simulink model "BrakeController_MBD"  (R2021b)
settings: Solver=FixedStepAuto  StartTime=0.0  StopTime=10.0  FixedStep=Ts  RelTol=1e-3
model workspace (MAT data in the model file):
  BrakePressure_Max = Simulink.Parameter
  BrakePressure_Max.Value = 100
  BrakePressure_Max.DataType = 'auto'
  BrakePressure_Max.Complexity = 'real'
  BrakePressure_Max.Dimensions = [1 1]
  Ts = Simulink.Parameter
  Ts.Value = 0.01
  Ts.DataType = 'auto'
  Ts.Complexity = 'real'
  Ts.Dimensions = [1 1]
  k = Simulink.Parameter
  k.Value = 2
  k.DataType = 'auto'
  k.Complexity = 'real'
  k.Dimensions = [1 1]
undefined symbols (not defined in the file): BrakeRequest, VehicleSpeed
settings Model: Creator=QNH2KOR  LastModifiedBy=QNH2KOR

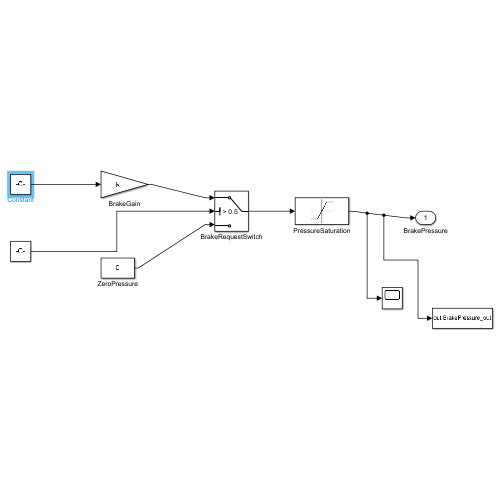
[thumbnail: Simulink's stored preview of the top-level diagram]
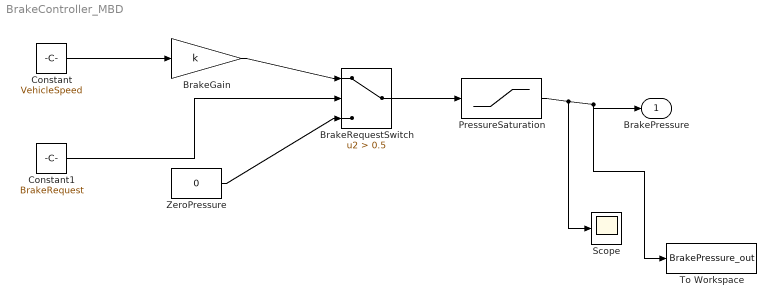
== system BrakeController_MBD ==
  BrakeGain : Gain  Gain=k
  BrakeRequestSwitch : Switch  Criteria=u2 > Threshold  Threshold=0.5
  Constant : Constant  Value=VehicleSpeed
  Constant1 : Constant  Value=BrakeRequest
  PressureSaturation : Saturate  UpperLimit=BrakePressure_Max  LowerLimit=0
  Scope : Scope
  To Workspace : ToWorkspace  VariableName=BrakePressure_out  SaveFormat=Timeseries  SampleTime=-1
  ZeroPressure : Constant  Value=0
  BrakePressure : Outport
  wires:
  Constant/1 -> BrakeGain/1
  BrakeGain/1 -> BrakeRequestSwitch/1
  Constant1/1 -> BrakeRequestSwitch/2
  ZeroPressure/1 -> BrakeRequestSwitch/3
  BrakeRequestSwitch/1 -> PressureSaturation/1
  PressureSaturation/1 -> Scope/1, To Workspace/1, BrakePressure/1
